simulink model "single_phase_multilevel_sm"  (R2026a)
settings: Solver=ode1be  StopTime=simlength  FixedStep=tc
values from neighbouring files (symbols this model uses):
  Vfc1_base = Udc/5    [plotting_modulation.m]    (also in plotting_results.m; plotting_results_hf.m)
  Vfc2_base = 2*Vfc1_base    [plotting_modulation.m]    (also in plotting_results.m; plotting_results_hf.m)
  Vfc3_base = 3*Vfc1_base    [plotting_modulation.m]    (also in plotting_results.m; plotting_results_hf.m)
  Vfc4_base = 4*Vfc1_base    [plotting_modulation.m]    (also in plotting_results.m; plotting_results_hf.m)
undefined symbols (not defined in the file or in its folder): g0_4Hz, g1_4Hz, I_FS, kalman_omega, kalman_theta, ki_i_inv, ki_v_inv, kp_i_inv, kp_v_inv, Lconn, LFu1, m_dead_time, m_duty_open_loop, magnitude, n1, n10, omega_ref, phase_shift_mod11, phase_shift_mod21, phase_shift_mod31, phase_shift_mod41, phase_shift_mod51, precharge_off, q1kalman, q2kalman, Rbalance, Rconn, RFu, Rkalman, RLFu1, tc, time_pwm_enable, tPWM, ts, V_FS, VCFc_5_init, Vgate_base
libraries: fl_lib x103, nesl_utility x61, simulink x1
(part 2 of 3)

== system single_phase_multilevel_sm/flying_capacitor_leg/fc1 ==
  CFc_1 : fl_lib/Electrical/Electrical Elements/Capacitor  c=CFc_1 F  r=1e-6 Ohm  g=0 1/Ohm  i_specify=off  i_priority=None  i=0 A  i_nominal_specify=off  i_nominal_value=1  i_nominal_unit=A  v_specify=off  v_priority=None  v=0 V  v_nominal_specify=off  v_nominal_value=1  v_nominal_unit=V  vc_specify=on  vc_priority=High  vc=VCFc_1_init V  vc_nominal_specify=off  vc_nominal_value=1  vc_nominal_unit=V
  CFi_HF_1 : fl_lib/Electrical/Electrical Elements/Capacitor  c=CFi_HF_1 F  r=1e-6 Ohm  g=0 1/Ohm  i_specify=off  i_priority=None  i=0 A  i_nominal_specify=off  i_nominal_value=1  i_nominal_unit=A  v_specify=off  v_priority=None  v=0 V  v_nominal_specify=off  v_nominal_value=1  v_nominal_unit=V  vc_specify=on  vc_priority=High  vc=VCFc_1_init V  vc_nominal_specify=off  vc_nominal_value=1  vc_nominal_unit=V
  Current Sensor : fl_lib/Electrical/Electrical Sensors/Current Sensor
  Current Sensor1 : fl_lib/Electrical/Electrical Sensors/Current Sensor
  PS-Simulink Converter : nesl_utility/PS-Simulink Converter  PhysicalDomain=network_engine_domain  SubClassName=ps_output  LeftPortType=input  RightPortType=output  PseudoPeriodic=off  Frequencies=[]  VectorFormat=1-D array  Unit=A  AffineConversion=off
  PS-Simulink Converter1 : nesl_utility/PS-Simulink Converter  PhysicalDomain=network_engine_domain  SubClassName=ps_output  LeftPortType=input  RightPortType=output  PseudoPeriodic=off  Frequencies=[]  VectorFormat=1-D array  Unit=V  AffineConversion=off
  PS-Simulink Converter2 : nesl_utility/PS-Simulink Converter  PhysicalDomain=network_engine_domain  SubClassName=ps_output  LeftPortType=input  RightPortType=output  PseudoPeriodic=off  Frequencies=[]  VectorFormat=1-D array  Unit=A  AffineConversion=off
  Voltage Sensor : fl_lib/Electrical/Electrical Sensors/Voltage Sensor
  1 : PMIOPort  Side=Left
  2 : PMIOPort  Port=2  Side=Right
  tag scope: current_flying_capacitor_1=global, current_hf_capacitor_1=global, voltage_flying_capacitor_1=global
  wires:
  PS-Simulink Converter1/1 -> [voltage_flying_capacitor_1]
  PS-Simulink Converter/1 -> [current_flying_capacitor_1]
  PS-Simulink Converter2/1 -> [current_hf_capacitor_1]
  connections:
  Current Sensor/RConn2 -- CFc_1/LConn1
  Voltage Sensor/RConn1 -- PS-Simulink Converter1/LConn1
  Current Sensor/RConn1 -- PS-Simulink Converter/LConn1
  Current Sensor/LConn1 -- Current Sensor1/LConn1 -- 1/RConn1 -- Voltage Sensor/LConn1
  Voltage Sensor/RConn2 -- 2/RConn1 -- CFc_1/RConn1 -- CFi_HF_1/RConn1
  Current Sensor1/RConn2 -- CFi_HF_1/LConn1
  Current Sensor1/RConn1 -- PS-Simulink Converter2/LConn1

== system single_phase_multilevel_sm/flying_capacitor_leg/fc2 ==
  CFc_2 : fl_lib/Electrical/Electrical Elements/Capacitor  c=CFc_2 F  r=1e-6 Ohm  g=0 1/Ohm  i_specify=off  i_priority=None  i=0 A  i_nominal_specify=off  i_nominal_value=1  i_nominal_unit=A  v_specify=off  v_priority=None  v=0 V  v_nominal_specify=off  v_nominal_value=1  v_nominal_unit=V  vc_specify=on  vc_priority=High  vc=VCFc_2_init V  vc_nominal_specify=off  vc_nominal_value=1  vc_nominal_unit=V
  CFi_HF_2 : fl_lib/Electrical/Electrical Elements/Capacitor  c=CFi_HF_2 F  r=1e-6 Ohm  g=0 1/Ohm  i_specify=off  i_priority=None  i=0 A  i_nominal_specify=off  i_nominal_value=1  i_nominal_unit=A  v_specify=off  v_priority=None  v=0 V  v_nominal_specify=off  v_nominal_value=1  v_nominal_unit=V  vc_specify=on  vc_priority=High  vc=VCFc_2_init V  vc_nominal_specify=off  vc_nominal_value=1  vc_nominal_unit=V
  Current Sensor : fl_lib/Electrical/Electrical Sensors/Current Sensor
  PS-Simulink Converter : nesl_utility/PS-Simulink Converter  PhysicalDomain=network_engine_domain  SubClassName=ps_output  LeftPortType=input  RightPortType=output  PseudoPeriodic=off  Frequencies=[]  VectorFormat=1-D array  Unit=A  AffineConversion=off
  PS-Simulink Converter2 : nesl_utility/PS-Simulink Converter  PhysicalDomain=network_engine_domain  SubClassName=ps_output  LeftPortType=input  RightPortType=output  PseudoPeriodic=off  Frequencies=[]  VectorFormat=1-D array  Unit=V  AffineConversion=off
  Voltage Sensor1 : fl_lib/Electrical/Electrical Sensors/Voltage Sensor
  1 : PMIOPort  Side=Left
  2 : PMIOPort  Port=2  Side=Right
  tag scope: current_flying_capacitor_2=global, voltage_flying_capacitor_2=global
  wires:
  PS-Simulink Converter2/1 -> [voltage_flying_capacitor_2]
  PS-Simulink Converter/1 -> [current_flying_capacitor_2]
  connections:
  Voltage Sensor1/LConn1 -- CFi_HF_2/LConn1 -- CFc_2/LConn1 -- 1/RConn1
  Voltage Sensor1/RConn1 -- PS-Simulink Converter2/LConn1
  Current Sensor/RConn1 -- PS-Simulink Converter/LConn1
  CFc_2/RConn1 -- Current Sensor/LConn1
  Voltage Sensor1/RConn2 -- CFi_HF_2/RConn1 -- Current Sensor/RConn2 -- 2/RConn1

== system single_phase_multilevel_sm/flying_capacitor_leg/fc3 ==
  CFc_3 : fl_lib/Electrical/Electrical Elements/Capacitor  c=CFc_3 F  r=1e-6 Ohm  g=0 1/Ohm  i_specify=off  i_priority=None  i=0 A  i_nominal_specify=off  i_nominal_value=1  i_nominal_unit=A  v_specify=off  v_priority=None  v=0 V  v_nominal_specify=off  v_nominal_value=1  v_nominal_unit=V  vc_specify=on  vc_priority=High  vc=VCFc_3_init V  vc_nominal_specify=off  vc_nominal_value=1  vc_nominal_unit=V
  CFi_HF_3 : fl_lib/Electrical/Electrical Elements/Capacitor  c=CFi_HF_3 F  r=1e-6 Ohm  g=0 1/Ohm  i_specify=off  i_priority=None  i=0 A  i_nominal_specify=off  i_nominal_value=1  i_nominal_unit=A  v_specify=off  v_priority=None  v=0 V  v_nominal_specify=off  v_nominal_value=1  v_nominal_unit=V  vc_specify=on  vc_priority=High  vc=VCFc_3_init V  vc_nominal_specify=off  vc_nominal_value=1  vc_nominal_unit=V
  Current Sensor : fl_lib/Electrical/Electrical Sensors/Current Sensor
  PS-Simulink Converter : nesl_utility/PS-Simulink Converter  PhysicalDomain=network_engine_domain  SubClassName=ps_output  LeftPortType=input  RightPortType=output  PseudoPeriodic=off  Frequencies=[]  VectorFormat=1-D array  Unit=A  AffineConversion=off
  PS-Simulink Converter2 : nesl_utility/PS-Simulink Converter  PhysicalDomain=network_engine_domain  SubClassName=ps_output  LeftPortType=input  RightPortType=output  PseudoPeriodic=off  Frequencies=[]  VectorFormat=1-D array  Unit=V  AffineConversion=off
  Voltage Sensor1 : fl_lib/Electrical/Electrical Sensors/Voltage Sensor
  1 : PMIOPort  Side=Left
  2 : PMIOPort  Port=2  Side=Right
  tag scope: current_flying_capacitor_3=global, voltage_flying_capacitor_3=global
  wires:
  PS-Simulink Converter2/1 -> [voltage_flying_capacitor_3]
  PS-Simulink Converter/1 -> [current_flying_capacitor_3]
  connections:
  CFc_3/LConn1 -- CFi_HF_3/LConn1 -- Voltage Sensor1/LConn1 -- 1/RConn1
  Voltage Sensor1/RConn1 -- PS-Simulink Converter2/LConn1
  Voltage Sensor1/RConn2 -- CFi_HF_3/RConn1 -- Current Sensor/RConn2 -- 2/RConn1
  Current Sensor/RConn1 -- PS-Simulink Converter/LConn1
  Current Sensor/LConn1 -- CFc_3/RConn1

== system single_phase_multilevel_sm/flying_capacitor_leg/fc4 ==
  CFc_4 : fl_lib/Electrical/Electrical Elements/Capacitor  c=CFc_4 F  r=1e-6 Ohm  g=0 1/Ohm  i_specify=off  i_priority=None  i=0 A  i_nominal_specify=off  i_nominal_value=1  i_nominal_unit=A  v_specify=off  v_priority=None  v=0 V  v_nominal_specify=off  v_nominal_value=1  v_nominal_unit=V  vc_specify=on  vc_priority=High  vc=VCFc_4_init V  vc_nominal_specify=off  vc_nominal_value=1  vc_nominal_unit=V
  CFi_HF_4 : fl_lib/Electrical/Electrical Elements/Capacitor  c=CFi_HF_4 F  r=1e-6 Ohm  g=0 1/Ohm  i_specify=off  i_priority=None  i=0 A  i_nominal_specify=off  i_nominal_value=1  i_nominal_unit=A  v_specify=off  v_priority=None  v=0 V  v_nominal_specify=off  v_nominal_value=1  v_nominal_unit=V  vc_specify=on  vc_priority=High  vc=VCFc_4_init V  vc_nominal_specify=off  vc_nominal_value=1  vc_nominal_unit=V
  Current Sensor : fl_lib/Electrical/Electrical Sensors/Current Sensor
  PS-Simulink Converter : nesl_utility/PS-Simulink Converter  PhysicalDomain=network_engine_domain  SubClassName=ps_output  LeftPortType=input  RightPortType=output  PseudoPeriodic=off  Frequencies=[]  VectorFormat=1-D array  Unit=A  AffineConversion=off
  PS-Simulink Converter2 : nesl_utility/PS-Simulink Converter  PhysicalDomain=network_engine_domain  SubClassName=ps_output  LeftPortType=input  RightPortType=output  PseudoPeriodic=off  Frequencies=[]  VectorFormat=1-D array  Unit=V  AffineConversion=off
  Voltage Sensor1 : fl_lib/Electrical/Electrical Sensors/Voltage Sensor
  1 : PMIOPort  Side=Left
  2 : PMIOPort  Port=2  Side=Right
  tag scope: current_flying_capacitor_4=global, voltage_flying_capacitor_4=global
  wires:
  PS-Simulink Converter2/1 -> [voltage_flying_capacitor_4]
  PS-Simulink Converter/1 -> [current_flying_capacitor_4]
  connections:
  Voltage Sensor1/LConn1 -- CFi_HF_4/LConn1 -- CFc_4/LConn1 -- 1/RConn1
  Voltage Sensor1/RConn1 -- PS-Simulink Converter2/LConn1
  Voltage Sensor1/RConn2 -- CFi_HF_4/RConn1 -- Current Sensor/RConn2 -- 2/RConn1
  Current Sensor/RConn1 -- PS-Simulink Converter/LConn1
  Current Sensor/LConn1 -- CFc_4/RConn1

== system single_phase_multilevel_sm/flying_capacitor_leg/fc51 ==
  CFc_51 : fl_lib/Electrical/Electrical Elements/Capacitor  c=CFc_51 F  r=1e-6 Ohm  g=0 1/Ohm  i_specify=off  i_priority=None  i=0 A  i_nominal_specify=off  i_nominal_value=1  i_nominal_unit=A  v_specify=off  v_priority=None  v=0 V  v_nominal_specify=off  v_nominal_value=1  v_nominal_unit=V  vc_specify=on  vc_priority=High  vc=VCFc_5_init/2 V  vc_nominal_specify=off  vc_nominal_value=1  vc_nominal_unit=V
  Current Sensor : fl_lib/Electrical/Electrical Sensors/Current Sensor
  PS-Simulink Converter : nesl_utility/PS-Simulink Converter  PhysicalDomain=network_engine_domain  SubClassName=ps_output  LeftPortType=input  RightPortType=output  PseudoPeriodic=off  Frequencies=[]  VectorFormat=1-D array  Unit=A  AffineConversion=off
  PS-Simulink Converter2 : nesl_utility/PS-Simulink Converter  PhysicalDomain=network_engine_domain  SubClassName=ps_output  LeftPortType=input  RightPortType=output  PseudoPeriodic=off  Frequencies=[]  VectorFormat=1-D array  Unit=V  AffineConversion=off
  Voltage Sensor1 : fl_lib/Electrical/Electrical Sensors/Voltage Sensor
  1 : PMIOPort  Side=Left
  2 : PMIOPort  Port=2  Side=Right
  tag scope: current_flying_capacitor_51=global, voltage_flying_capacitor_51=global
  wires:
  PS-Simulink Converter/1 -> [current_flying_capacitor_51]
  PS-Simulink Converter2/1 -> [voltage_flying_capacitor_51]
  connections:
  CFc_51/LConn1 -- Voltage Sensor1/LConn1 -- 1/RConn1
  Current Sensor/RConn1 -- PS-Simulink Converter/LConn1
  Current Sensor/LConn1 -- CFc_51/RConn1
  Current Sensor/RConn2 -- Voltage Sensor1/RConn2 -- 2/RConn1
  Voltage Sensor1/RConn1 -- PS-Simulink Converter2/LConn1

== system single_phase_multilevel_sm/flying_capacitor_leg/fc52 ==
  CFc_52 : fl_lib/Electrical/Electrical Elements/Capacitor  c=CFc_52 F  r=1e-6 Ohm  g=0 1/Ohm  i_specify=off  i_priority=None  i=0 A  i_nominal_specify=off  i_nominal_value=1  i_nominal_unit=A  v_specify=off  v_priority=None  v=0 V  v_nominal_specify=off  v_nominal_value=1  v_nominal_unit=V  vc_specify=on  vc_priority=High  vc=VCFc_5_init/2 V  vc_nominal_specify=off  vc_nominal_value=1  vc_nominal_unit=V
  Current Sensor : fl_lib/Electrical/Electrical Sensors/Current Sensor
  PS-Simulink Converter : nesl_utility/PS-Simulink Converter  PhysicalDomain=network_engine_domain  SubClassName=ps_output  LeftPortType=input  RightPortType=output  PseudoPeriodic=off  Frequencies=[]  VectorFormat=1-D array  Unit=A  AffineConversion=off
  PS-Simulink Converter2 : nesl_utility/PS-Simulink Converter  PhysicalDomain=network_engine_domain  SubClassName=ps_output  LeftPortType=input  RightPortType=output  PseudoPeriodic=off  Frequencies=[]  VectorFormat=1-D array  Unit=V  AffineConversion=off
  Voltage Sensor1 : fl_lib/Electrical/Electrical Sensors/Voltage Sensor
  1 : PMIOPort  Side=Left
  2 : PMIOPort  Port=2  Side=Right
  tag scope: current_flying_capacitor_52=global, voltage_flying_capacitor_52=global
  wires:
  PS-Simulink Converter/1 -> [current_flying_capacitor_52]
  PS-Simulink Converter2/1 -> [voltage_flying_capacitor_52]
  connections:
  CFc_52/LConn1 -- Voltage Sensor1/LConn1 -- 1/RConn1
  Current Sensor/RConn1 -- PS-Simulink Converter/LConn1
  Current Sensor/RConn2 -- Voltage Sensor1/RConn2 -- 2/RConn1
  CFc_52/RConn1 -- Current Sensor/LConn1
  Voltage Sensor1/RConn1 -- PS-Simulink Converter2/LConn1

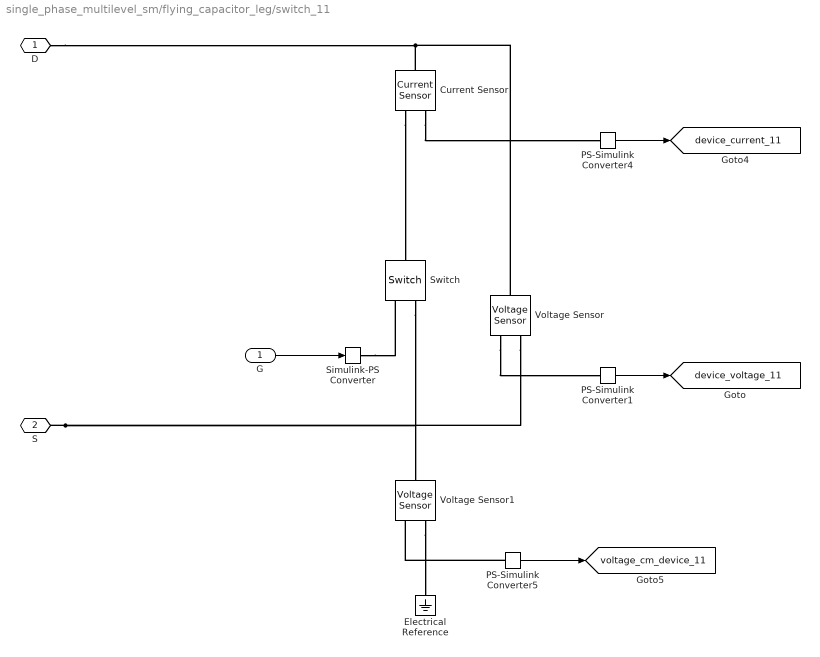
== system single_phase_multilevel_sm/flying_capacitor_leg/switch_11 ==
  G : Inport
  Current Sensor : fl_lib/Electrical/Electrical Sensors/Current Sensor
  Electrical Reference : fl_lib/Electrical/Electrical Elements/Electrical Reference
  PS-Simulink Converter1 : nesl_utility/PS-Simulink Converter  PhysicalDomain=network_engine_domain  SubClassName=ps_output  LeftPortType=input  RightPortType=output  PseudoPeriodic=off  Frequencies=[]  VectorFormat=1-D array  Unit=V  AffineConversion=off
  PS-Simulink Converter4 : nesl_utility/PS-Simulink Converter  PhysicalDomain=network_engine_domain  SubClassName=ps_output  LeftPortType=input  RightPortType=output  PseudoPeriodic=off  Frequencies=[]  VectorFormat=1-D array  Unit=A  AffineConversion=off
  PS-Simulink Converter5 : nesl_utility/PS-Simulink Converter  PhysicalDomain=network_engine_domain  SubClassName=ps_output  LeftPortType=input  RightPortType=output  PseudoPeriodic=off  Frequencies=[]  VectorFormat=1-D array  Unit=V  AffineConversion=off
  Simulink-PS Converter : nesl_utility/Simulink-PS Converter  PhysicalDomain=network_engine_domain  SubClassName=ps_input  LeftPortType=input  RightPortType=output  PseudoPeriodic=off  Frequencies=[]  NoiseDistribution=none  NoiseParameters=[]  Unit=V  AffineConversion=off  FilteringAndDerivatives=provide  SimscapeFilterOrder=1  InputFilterTimeConstant=0.001  UdotUserProvided=0
  Switch : fl_lib/Electrical/Electrical Elements/Switch  R_closed=1e-3 Ohm  G_open=1e-8 1/Ohm  Threshold=3  i_specify=off  i_priority=None  i=0 A  i_nominal_specify=off  i_nominal_value=1  i_nominal_unit=A  v_specify=off  v_priority=None  v=0 V  v_nominal_specify=off  v_nominal_value=1  v_nominal_unit=V
  Voltage Sensor : fl_lib/Electrical/Electrical Sensors/Voltage Sensor
  Voltage Sensor1 : fl_lib/Electrical/Electrical Sensors/Voltage Sensor
  D : PMIOPort  Side=Left
  S : PMIOPort  Port=2  Side=Right
  tag scope: device_current_11=global, device_voltage_11=global, voltage_cm_device_11=global
  wires:
  PS-Simulink Converter1/1 -> [device_voltage_11]
  PS-Simulink Converter4/1 -> [device_current_11]
  PS-Simulink Converter5/1 -> [voltage_cm_device_11]
  G/1 -> Simulink-PS Converter/1
  connections:
  Voltage Sensor/RConn1 -- PS-Simulink Converter1/LConn1
  S/RConn1 -- Switch/RConn2 -- Voltage Sensor/RConn2 -- Voltage Sensor1/LConn1
  Current Sensor/LConn1 -- D/RConn1 -- Voltage Sensor/LConn1
  Current Sensor/RConn1 -- PS-Simulink Converter4/LConn1
  PS-Simulink Converter5/LConn1 -- Voltage Sensor1/RConn1
  Voltage Sensor1/RConn2 -- Electrical Reference/LConn1
  Simulink-PS Converter/RConn1 -- Switch/RConn1
  Current Sensor/RConn2 -- Switch/LConn1

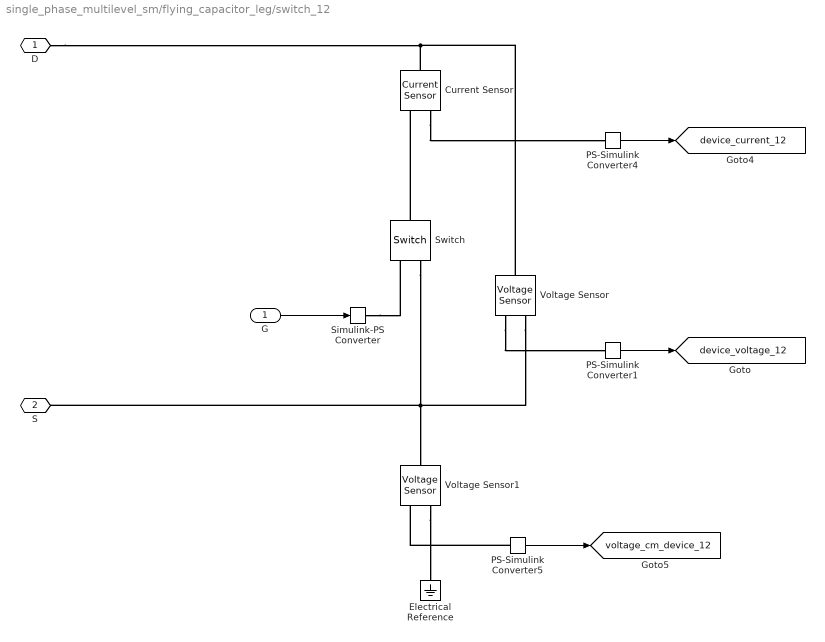
== system single_phase_multilevel_sm/flying_capacitor_leg/switch_12 ==
  G : Inport
  Current Sensor : fl_lib/Electrical/Electrical Sensors/Current Sensor
  Electrical Reference : fl_lib/Electrical/Electrical Elements/Electrical Reference
  PS-Simulink Converter1 : nesl_utility/PS-Simulink Converter  PhysicalDomain=network_engine_domain  SubClassName=ps_output  LeftPortType=input  RightPortType=output  PseudoPeriodic=off  Frequencies=[]  VectorFormat=1-D array  Unit=V  AffineConversion=off
  PS-Simulink Converter4 : nesl_utility/PS-Simulink Converter  PhysicalDomain=network_engine_domain  SubClassName=ps_output  LeftPortType=input  RightPortType=output  PseudoPeriodic=off  Frequencies=[]  VectorFormat=1-D array  Unit=A  AffineConversion=off
  PS-Simulink Converter5 : nesl_utility/PS-Simulink Converter  PhysicalDomain=network_engine_domain  SubClassName=ps_output  LeftPortType=input  RightPortType=output  PseudoPeriodic=off  Frequencies=[]  VectorFormat=1-D array  Unit=V  AffineConversion=off
  Simulink-PS Converter : nesl_utility/Simulink-PS Converter  PhysicalDomain=network_engine_domain  SubClassName=ps_input  LeftPortType=input  RightPortType=output  PseudoPeriodic=off  Frequencies=[]  NoiseDistribution=none  NoiseParameters=[]  Unit=V  AffineConversion=off  FilteringAndDerivatives=provide  SimscapeFilterOrder=1  InputFilterTimeConstant=0.001  UdotUserProvided=0
  Switch : fl_lib/Electrical/Electrical Elements/Switch  R_closed=1e-3 Ohm  G_open=1e-8 1/Ohm  Threshold=3  i_specify=off  i_priority=None  i=0 A  i_nominal_specify=off  i_nominal_value=1  i_nominal_unit=A  v_specify=off  v_priority=None  v=0 V  v_nominal_specify=off  v_nominal_value=1  v_nominal_unit=V
  Voltage Sensor : fl_lib/Electrical/Electrical Sensors/Voltage Sensor
  Voltage Sensor1 : fl_lib/Electrical/Electrical Sensors/Voltage Sensor
  D : PMIOPort  Side=Left
  S : PMIOPort  Port=2  Side=Right
  tag scope: device_current_12=global, device_voltage_12=global, voltage_cm_device_12=global
  wires:
  PS-Simulink Converter1/1 -> [device_voltage_12]
  PS-Simulink Converter4/1 -> [device_current_12]
  PS-Simulink Converter5/1 -> [voltage_cm_device_12]
  G/1 -> Simulink-PS Converter/1
  connections:
  Voltage Sensor/RConn2 -- S/RConn1 -- Switch/RConn2 -- Voltage Sensor1/LConn1
  Voltage Sensor/RConn1 -- PS-Simulink Converter1/LConn1
  Current Sensor/LConn1 -- D/RConn1 -- Voltage Sensor/LConn1
  Current Sensor/RConn1 -- PS-Simulink Converter4/LConn1
  PS-Simulink Converter5/LConn1 -- Voltage Sensor1/RConn1
  Voltage Sensor1/RConn2 -- Electrical Reference/LConn1
  Simulink-PS Converter/RConn1 -- Switch/RConn1
  Switch/LConn1 -- Current Sensor/RConn2

== system single_phase_multilevel_sm/flying_capacitor_leg/switch_21 ==
  G : Inport
  Current Sensor : fl_lib/Electrical/Electrical Sensors/Current Sensor
  Electrical Reference : fl_lib/Electrical/Electrical Elements/Electrical Reference
  PS-Simulink Converter1 : nesl_utility/PS-Simulink Converter  PhysicalDomain=network_engine_domain  SubClassName=ps_output  LeftPortType=input  RightPortType=output  PseudoPeriodic=off  Frequencies=[]  VectorFormat=1-D array  Unit=V  AffineConversion=off
  PS-Simulink Converter4 : nesl_utility/PS-Simulink Converter  PhysicalDomain=network_engine_domain  SubClassName=ps_output  LeftPortType=input  RightPortType=output  PseudoPeriodic=off  Frequencies=[]  VectorFormat=1-D array  Unit=A  AffineConversion=off
  PS-Simulink Converter5 : nesl_utility/PS-Simulink Converter  PhysicalDomain=network_engine_domain  SubClassName=ps_output  LeftPortType=input  RightPortType=output  PseudoPeriodic=off  Frequencies=[]  VectorFormat=1-D array  Unit=V  AffineConversion=off
  Simulink-PS Converter : nesl_utility/Simulink-PS Converter  PhysicalDomain=network_engine_domain  SubClassName=ps_input  LeftPortType=input  RightPortType=output  PseudoPeriodic=off  Frequencies=[]  NoiseDistribution=none  NoiseParameters=[]  Unit=V  AffineConversion=off  FilteringAndDerivatives=provide  SimscapeFilterOrder=1  InputFilterTimeConstant=0.001  UdotUserProvided=0
  Switch : fl_lib/Electrical/Electrical Elements/Switch  R_closed=1e-3 Ohm  G_open=1e-8 1/Ohm  Threshold=3  i_specify=off  i_priority=None  i=0 A  i_nominal_specify=off  i_nominal_value=1  i_nominal_unit=A  v_specify=off  v_priority=None  v=0 V  v_nominal_specify=off  v_nominal_value=1  v_nominal_unit=V
  Voltage Sensor : fl_lib/Electrical/Electrical Sensors/Voltage Sensor
  Voltage Sensor1 : fl_lib/Electrical/Electrical Sensors/Voltage Sensor
  D : PMIOPort  Side=Left
  S : PMIOPort  Port=2  Side=Right
  tag scope: device_current_21=global, device_voltage_21=global, voltage_cm_device_21=global
  wires:
  PS-Simulink Converter1/1 -> [device_voltage_21]
  PS-Simulink Converter4/1 -> [device_current_21]
  PS-Simulink Converter5/1 -> [voltage_cm_device_21]
  G/1 -> Simulink-PS Converter/1
  connections:
  Voltage Sensor/RConn2 -- Switch/RConn2 -- S/RConn1 -- Voltage Sensor1/LConn1
  Voltage Sensor/RConn1 -- PS-Simulink Converter1/LConn1
  Current Sensor/LConn1 -- Voltage Sensor/LConn1 -- D/RConn1
  Current Sensor/RConn1 -- PS-Simulink Converter4/LConn1
  PS-Simulink Converter5/LConn1 -- Voltage Sensor1/RConn1
  Voltage Sensor1/RConn2 -- Electrical Reference/LConn1
  Simulink-PS Converter/RConn1 -- Switch/RConn1
  Current Sensor/RConn2 -- Switch/LConn1

== system single_phase_multilevel_sm/flying_capacitor_leg/switch_22 ==
  G : Inport
  Current Sensor : fl_lib/Electrical/Electrical Sensors/Current Sensor
  Electrical Reference : fl_lib/Electrical/Electrical Elements/Electrical Reference
  PS-Simulink Converter1 : nesl_utility/PS-Simulink Converter  PhysicalDomain=network_engine_domain  SubClassName=ps_output  LeftPortType=input  RightPortType=output  PseudoPeriodic=off  Frequencies=[]  VectorFormat=1-D array  Unit=V  AffineConversion=off
  PS-Simulink Converter4 : nesl_utility/PS-Simulink Converter  PhysicalDomain=network_engine_domain  SubClassName=ps_output  LeftPortType=input  RightPortType=output  PseudoPeriodic=off  Frequencies=[]  VectorFormat=1-D array  Unit=A  AffineConversion=off
  PS-Simulink Converter5 : nesl_utility/PS-Simulink Converter  PhysicalDomain=network_engine_domain  SubClassName=ps_output  LeftPortType=input  RightPortType=output  PseudoPeriodic=off  Frequencies=[]  VectorFormat=1-D array  Unit=V  AffineConversion=off
  Simulink-PS Converter : nesl_utility/Simulink-PS Converter  PhysicalDomain=network_engine_domain  SubClassName=ps_input  LeftPortType=input  RightPortType=output  PseudoPeriodic=off  Frequencies=[]  NoiseDistribution=none  NoiseParameters=[]  Unit=V  AffineConversion=off  FilteringAndDerivatives=provide  SimscapeFilterOrder=1  InputFilterTimeConstant=0.001  UdotUserProvided=0
  Switch : fl_lib/Electrical/Electrical Elements/Switch  R_closed=1e-3 Ohm  G_open=1e-8 1/Ohm  Threshold=3  i_specify=off  i_priority=None  i=0 A  i_nominal_specify=off  i_nominal_value=1  i_nominal_unit=A  v_specify=off  v_priority=None  v=0 V  v_nominal_specify=off  v_nominal_value=1  v_nominal_unit=V
  Voltage Sensor : fl_lib/Electrical/Electrical Sensors/Voltage Sensor
  Voltage Sensor1 : fl_lib/Electrical/Electrical Sensors/Voltage Sensor
  D : PMIOPort  Side=Left
  S : PMIOPort  Port=2  Side=Right
  tag scope: device_current_22=global, device_voltage_22=global, voltage_cm_device_22=global
  wires:
  PS-Simulink Converter1/1 -> [device_voltage_22]
  PS-Simulink Converter4/1 -> [device_current_22]
  PS-Simulink Converter5/1 -> [voltage_cm_device_22]
  G/1 -> Simulink-PS Converter/1
  connections:
  Voltage Sensor/RConn1 -- PS-Simulink Converter1/LConn1
  S/RConn1 -- Switch/RConn2 -- Voltage Sensor/RConn2 -- Voltage Sensor1/LConn1
  Current Sensor/LConn1 -- Voltage Sensor/LConn1 -- D/RConn1
  Current Sensor/RConn1 -- PS-Simulink Converter4/LConn1
  PS-Simulink Converter5/LConn1 -- Voltage Sensor1/RConn1
  Voltage Sensor1/RConn2 -- Electrical Reference/LConn1
  Simulink-PS Converter/RConn1 -- Switch/RConn1
  Switch/LConn1 -- Current Sensor/RConn2

== system single_phase_multilevel_sm/flying_capacitor_leg/switch_31 ==
  G : Inport
  Current Sensor : fl_lib/Electrical/Electrical Sensors/Current Sensor
  Electrical Reference : fl_lib/Electrical/Electrical Elements/Electrical Reference
  PS-Simulink Converter1 : nesl_utility/PS-Simulink Converter  PhysicalDomain=network_engine_domain  SubClassName=ps_output  LeftPortType=input  RightPortType=output  PseudoPeriodic=off  Frequencies=[]  VectorFormat=1-D array  Unit=V  AffineConversion=off
  PS-Simulink Converter4 : nesl_utility/PS-Simulink Converter  PhysicalDomain=network_engine_domain  SubClassName=ps_output  LeftPortType=input  RightPortType=output  PseudoPeriodic=off  Frequencies=[]  VectorFormat=1-D array  Unit=A  AffineConversion=off
  PS-Simulink Converter5 : nesl_utility/PS-Simulink Converter  PhysicalDomain=network_engine_domain  SubClassName=ps_output  LeftPortType=input  RightPortType=output  PseudoPeriodic=off  Frequencies=[]  VectorFormat=1-D array  Unit=V  AffineConversion=off
  Simulink-PS Converter : nesl_utility/Simulink-PS Converter  PhysicalDomain=network_engine_domain  SubClassName=ps_input  LeftPortType=input  RightPortType=output  PseudoPeriodic=off  Frequencies=[]  NoiseDistribution=none  NoiseParameters=[]  Unit=V  AffineConversion=off  FilteringAndDerivatives=provide  SimscapeFilterOrder=1  InputFilterTimeConstant=0.001  UdotUserProvided=0
  Switch : fl_lib/Electrical/Electrical Elements/Switch  R_closed=1e-3 Ohm  G_open=1e-8 1/Ohm  Threshold=3  i_specify=off  i_priority=None  i=0 A  i_nominal_specify=off  i_nominal_value=1  i_nominal_unit=A  v_specify=off  v_priority=None  v=0 V  v_nominal_specify=off  v_nominal_value=1  v_nominal_unit=V
  Voltage Sensor : fl_lib/Electrical/Electrical Sensors/Voltage Sensor
  Voltage Sensor1 : fl_lib/Electrical/Electrical Sensors/Voltage Sensor
  D : PMIOPort  Side=Left
  S : PMIOPort  Port=2  Side=Right
  tag scope: device_current_31=global, device_voltage_31=global, voltage_cm_device_31=global
  wires:
  PS-Simulink Converter1/1 -> [device_voltage_31]
  PS-Simulink Converter4/1 -> [device_current_31]
  PS-Simulink Converter5/1 -> [voltage_cm_device_31]
  G/1 -> Simulink-PS Converter/1
  connections:
  Voltage Sensor/RConn1 -- PS-Simulink Converter1/LConn1
  S/RConn1 -- Switch/RConn2 -- Voltage Sensor/RConn2 -- Voltage Sensor1/LConn1
  Current Sensor/LConn1 -- Voltage Sensor/LConn1 -- D/RConn1
  Current Sensor/RConn1 -- PS-Simulink Converter4/LConn1
  PS-Simulink Converter5/LConn1 -- Voltage Sensor1/RConn1
  Voltage Sensor1/RConn2 -- Electrical Reference/LConn1
  Simulink-PS Converter/RConn1 -- Switch/RConn1
  Current Sensor/RConn2 -- Switch/LConn1

== system single_phase_multilevel_sm/flying_capacitor_leg/switch_32 ==
  G : Inport
  Current Sensor : fl_lib/Electrical/Electrical Sensors/Current Sensor
  Electrical Reference : fl_lib/Electrical/Electrical Elements/Electrical Reference
  PS-Simulink Converter1 : nesl_utility/PS-Simulink Converter  PhysicalDomain=network_engine_domain  SubClassName=ps_output  LeftPortType=input  RightPortType=output  PseudoPeriodic=off  Frequencies=[]  VectorFormat=1-D array  Unit=V  AffineConversion=off
  PS-Simulink Converter4 : nesl_utility/PS-Simulink Converter  PhysicalDomain=network_engine_domain  SubClassName=ps_output  LeftPortType=input  RightPortType=output  PseudoPeriodic=off  Frequencies=[]  VectorFormat=1-D array  Unit=A  AffineConversion=off
  PS-Simulink Converter5 : nesl_utility/PS-Simulink Converter  PhysicalDomain=network_engine_domain  SubClassName=ps_output  LeftPortType=input  RightPortType=output  PseudoPeriodic=off  Frequencies=[]  VectorFormat=1-D array  Unit=V  AffineConversion=off
  Simulink-PS Converter : nesl_utility/Simulink-PS Converter  PhysicalDomain=network_engine_domain  SubClassName=ps_input  LeftPortType=input  RightPortType=output  PseudoPeriodic=off  Frequencies=[]  NoiseDistribution=none  NoiseParameters=[]  Unit=V  AffineConversion=off  FilteringAndDerivatives=provide  SimscapeFilterOrder=1  InputFilterTimeConstant=0.001  UdotUserProvided=0
  Switch : fl_lib/Electrical/Electrical Elements/Switch  R_closed=1e-3 Ohm  G_open=1e-8 1/Ohm  Threshold=3  i_specify=off  i_priority=None  i=0 A  i_nominal_specify=off  i_nominal_value=1  i_nominal_unit=A  v_specify=off  v_priority=None  v=0 V  v_nominal_specify=off  v_nominal_value=1  v_nominal_unit=V
  Voltage Sensor : fl_lib/Electrical/Electrical Sensors/Voltage Sensor
  Voltage Sensor1 : fl_lib/Electrical/Electrical Sensors/Voltage Sensor
  D : PMIOPort  Side=Left
  S : PMIOPort  Port=2  Side=Right
  tag scope: device_current_32=global, device_voltage_32=global, voltage_cm_device_32=global
  wires:
  PS-Simulink Converter1/1 -> [device_voltage_32]
  PS-Simulink Converter4/1 -> [device_current_32]
  PS-Simulink Converter5/1 -> [voltage_cm_device_32]
  G/1 -> Simulink-PS Converter/1
  connections:
  Voltage Sensor/RConn2 -- Voltage Sensor1/LConn1 -- Switch/RConn2 -- S/RConn1
  Voltage Sensor/RConn1 -- PS-Simulink Converter1/LConn1
  Current Sensor/LConn1 -- D/RConn1 -- Voltage Sensor/LConn1
  Current Sensor/RConn1 -- PS-Simulink Converter4/LConn1
  PS-Simulink Converter5/LConn1 -- Voltage Sensor1/RConn1
  Voltage Sensor1/RConn2 -- Electrical Reference/LConn1
  Simulink-PS Converter/RConn1 -- Switch/RConn1
  Switch/LConn1 -- Current Sensor/RConn2

== system single_phase_multilevel_sm/flying_capacitor_leg/switch_41 ==
  G : Inport
  Current Sensor : fl_lib/Electrical/Electrical Sensors/Current Sensor
  Electrical Reference : fl_lib/Electrical/Electrical Elements/Electrical Reference
  PS-Simulink Converter1 : nesl_utility/PS-Simulink Converter  PhysicalDomain=network_engine_domain  SubClassName=ps_output  LeftPortType=input  RightPortType=output  PseudoPeriodic=off  Frequencies=[]  VectorFormat=1-D array  Unit=V  AffineConversion=off
  PS-Simulink Converter4 : nesl_utility/PS-Simulink Converter  PhysicalDomain=network_engine_domain  SubClassName=ps_output  LeftPortType=input  RightPortType=output  PseudoPeriodic=off  Frequencies=[]  VectorFormat=1-D array  Unit=A  AffineConversion=off
  PS-Simulink Converter5 : nesl_utility/PS-Simulink Converter  PhysicalDomain=network_engine_domain  SubClassName=ps_output  LeftPortType=input  RightPortType=output  PseudoPeriodic=off  Frequencies=[]  VectorFormat=1-D array  Unit=V  AffineConversion=off
  Simulink-PS Converter : nesl_utility/Simulink-PS Converter  PhysicalDomain=network_engine_domain  SubClassName=ps_input  LeftPortType=input  RightPortType=output  PseudoPeriodic=off  Frequencies=[]  NoiseDistribution=none  NoiseParameters=[]  Unit=V  AffineConversion=off  FilteringAndDerivatives=provide  SimscapeFilterOrder=1  InputFilterTimeConstant=0.001  UdotUserProvided=0
  Switch : fl_lib/Electrical/Electrical Elements/Switch  R_closed=1e-3 Ohm  G_open=1e-8 1/Ohm  Threshold=3  i_specify=off  i_priority=None  i=0 A  i_nominal_specify=off  i_nominal_value=1  i_nominal_unit=A  v_specify=off  v_priority=None  v=0 V  v_nominal_specify=off  v_nominal_value=1  v_nominal_unit=V
  Voltage Sensor : fl_lib/Electrical/Electrical Sensors/Voltage Sensor
  Voltage Sensor1 : fl_lib/Electrical/Electrical Sensors/Voltage Sensor
  D : PMIOPort  Side=Left
  S : PMIOPort  Port=2  Side=Right
  tag scope: device_current_41=global, device_voltage_41=global, voltage_cm_device_41=global
  wires:
  PS-Simulink Converter1/1 -> [device_voltage_41]
  PS-Simulink Converter4/1 -> [device_current_41]
  PS-Simulink Converter5/1 -> [voltage_cm_device_41]
  G/1 -> Simulink-PS Converter/1
  connections:
  Voltage Sensor/RConn2 -- Switch/RConn2 -- S/RConn1 -- Voltage Sensor1/LConn1
  Voltage Sensor/RConn1 -- PS-Simulink Converter1/LConn1
  Current Sensor/LConn1 -- Voltage Sensor/LConn1 -- D/RConn1
  Current Sensor/RConn1 -- PS-Simulink Converter4/LConn1
  PS-Simulink Converter5/LConn1 -- Voltage Sensor1/RConn1
  Voltage Sensor1/RConn2 -- Electrical Reference/LConn1
  Simulink-PS Converter/RConn1 -- Switch/RConn1
  Switch/LConn1 -- Current Sensor/RConn2

== system single_phase_multilevel_sm/flying_capacitor_leg/switch_42 ==
  G : Inport
  Current Sensor : fl_lib/Electrical/Electrical Sensors/Current Sensor
  Electrical Reference : fl_lib/Electrical/Electrical Elements/Electrical Reference
  PS-Simulink Converter1 : nesl_utility/PS-Simulink Converter  PhysicalDomain=network_engine_domain  SubClassName=ps_output  LeftPortType=input  RightPortType=output  PseudoPeriodic=off  Frequencies=[]  VectorFormat=1-D array  Unit=V  AffineConversion=off
  PS-Simulink Converter4 : nesl_utility/PS-Simulink Converter  PhysicalDomain=network_engine_domain  SubClassName=ps_output  LeftPortType=input  RightPortType=output  PseudoPeriodic=off  Frequencies=[]  VectorFormat=1-D array  Unit=A  AffineConversion=off
  PS-Simulink Converter5 : nesl_utility/PS-Simulink Converter  PhysicalDomain=network_engine_domain  SubClassName=ps_output  LeftPortType=input  RightPortType=output  PseudoPeriodic=off  Frequencies=[]  VectorFormat=1-D array  Unit=V  AffineConversion=off
  Simulink-PS Converter : nesl_utility/Simulink-PS Converter  PhysicalDomain=network_engine_domain  SubClassName=ps_input  LeftPortType=input  RightPortType=output  PseudoPeriodic=off  Frequencies=[]  NoiseDistribution=none  NoiseParameters=[]  Unit=V  AffineConversion=off  FilteringAndDerivatives=provide  SimscapeFilterOrder=1  InputFilterTimeConstant=0.001  UdotUserProvided=0
  Switch : fl_lib/Electrical/Electrical Elements/Switch  R_closed=1e-3 Ohm  G_open=1e-8 1/Ohm  Threshold=3  i_specify=off  i_priority=None  i=0 A  i_nominal_specify=off  i_nominal_value=1  i_nominal_unit=A  v_specify=off  v_priority=None  v=0 V  v_nominal_specify=off  v_nominal_value=1  v_nominal_unit=V
  Voltage Sensor : fl_lib/Electrical/Electrical Sensors/Voltage Sensor
  Voltage Sensor1 : fl_lib/Electrical/Electrical Sensors/Voltage Sensor
  D : PMIOPort  Side=Left
  S : PMIOPort  Port=2  Side=Right
  tag scope: device_current_42=global, device_voltage_42=global, voltage_cm_device_42=global
  wires:
  PS-Simulink Converter1/1 -> [device_voltage_42]
  PS-Simulink Converter4/1 -> [device_current_42]
  PS-Simulink Converter5/1 -> [voltage_cm_device_42]
  G/1 -> Simulink-PS Converter/1
  connections:
  Voltage Sensor/RConn1 -- PS-Simulink Converter1/LConn1
  S/RConn1 -- Voltage Sensor1/LConn1 -- Switch/RConn2 -- Voltage Sensor/RConn2
  Current Sensor/LConn1 -- Voltage Sensor/LConn1 -- D/RConn1
  Current Sensor/RConn1 -- PS-Simulink Converter4/LConn1
  PS-Simulink Converter5/LConn1 -- Voltage Sensor1/RConn1
  Voltage Sensor1/RConn2 -- Electrical Reference/LConn1
  Simulink-PS Converter/RConn1 -- Switch/RConn1
  Switch/LConn1 -- Current Sensor/RConn2

== system single_phase_multilevel_sm/flying_capacitor_leg/switch_51 ==
  G : Inport
  Current Sensor : fl_lib/Electrical/Electrical Sensors/Current Sensor
  Electrical Reference : fl_lib/Electrical/Electrical Elements/Electrical Reference
  PS-Simulink Converter1 : nesl_utility/PS-Simulink Converter  PhysicalDomain=network_engine_domain  SubClassName=ps_output  LeftPortType=input  RightPortType=output  PseudoPeriodic=off  Frequencies=[]  VectorFormat=1-D array  Unit=V  AffineConversion=off
  PS-Simulink Converter4 : nesl_utility/PS-Simulink Converter  PhysicalDomain=network_engine_domain  SubClassName=ps_output  LeftPortType=input  RightPortType=output  PseudoPeriodic=off  Frequencies=[]  VectorFormat=1-D array  Unit=A  AffineConversion=off
  PS-Simulink Converter5 : nesl_utility/PS-Simulink Converter  PhysicalDomain=network_engine_domain  SubClassName=ps_output  LeftPortType=input  RightPortType=output  PseudoPeriodic=off  Frequencies=[]  VectorFormat=1-D array  Unit=V  AffineConversion=off
  Simulink-PS Converter : nesl_utility/Simulink-PS Converter  PhysicalDomain=network_engine_domain  SubClassName=ps_input  LeftPortType=input  RightPortType=output  PseudoPeriodic=off  Frequencies=[]  NoiseDistribution=none  NoiseParameters=[]  Unit=V  AffineConversion=off  FilteringAndDerivatives=provide  SimscapeFilterOrder=1  InputFilterTimeConstant=0.001  UdotUserProvided=0
  Switch : fl_lib/Electrical/Electrical Elements/Switch  R_closed=1e-3 Ohm  G_open=1e-8 1/Ohm  Threshold=3  i_specify=off  i_priority=None  i=0 A  i_nominal_specify=off  i_nominal_value=1  i_nominal_unit=A  v_specify=off  v_priority=None  v=0 V  v_nominal_specify=off  v_nominal_value=1  v_nominal_unit=V
  Voltage Sensor : fl_lib/Electrical/Electrical Sensors/Voltage Sensor
  Voltage Sensor1 : fl_lib/Electrical/Electrical Sensors/Voltage Sensor
  D : PMIOPort  Side=Left
  S : PMIOPort  Port=2  Side=Right
  tag scope: device_current_51=global, device_voltage_51=global, voltage_cm_device_51=global
  wires:
  PS-Simulink Converter1/1 -> [device_voltage_51]
  PS-Simulink Converter4/1 -> [device_current_51]
  PS-Simulink Converter5/1 -> [voltage_cm_device_51]
  G/1 -> Simulink-PS Converter/1
  connections:
  Voltage Sensor/RConn1 -- PS-Simulink Converter1/LConn1
  D/RConn1 -- Voltage Sensor/LConn1 -- Current Sensor/LConn1
  Voltage Sensor/RConn2 -- Switch/RConn2 -- S/RConn1 -- Voltage Sensor1/LConn1
  Switch/LConn1 -- Current Sensor/RConn2
  Current Sensor/RConn1 -- PS-Simulink Converter4/LConn1
  Voltage Sensor1/RConn2 -- Electrical Reference/LConn1
  PS-Simulink Converter5/LConn1 -- Voltage Sensor1/RConn1
  Simulink-PS Converter/RConn1 -- Switch/RConn1

== system single_phase_multilevel_sm/flying_capacitor_leg/switch_52 ==
  G : Inport
  Current Sensor : fl_lib/Electrical/Electrical Sensors/Current Sensor
  Electrical Reference : fl_lib/Electrical/Electrical Elements/Electrical Reference
  PS-Simulink Converter1 : nesl_utility/PS-Simulink Converter  PhysicalDomain=network_engine_domain  SubClassName=ps_output  LeftPortType=input  RightPortType=output  PseudoPeriodic=off  Frequencies=[]  VectorFormat=1-D array  Unit=V  AffineConversion=off
  PS-Simulink Converter4 : nesl_utility/PS-Simulink Converter  PhysicalDomain=network_engine_domain  SubClassName=ps_output  LeftPortType=input  RightPortType=output  PseudoPeriodic=off  Frequencies=[]  VectorFormat=1-D array  Unit=A  AffineConversion=off
  PS-Simulink Converter5 : nesl_utility/PS-Simulink Converter  PhysicalDomain=network_engine_domain  SubClassName=ps_output  LeftPortType=input  RightPortType=output  PseudoPeriodic=off  Frequencies=[]  VectorFormat=1-D array  Unit=V  AffineConversion=off
  Simulink-PS Converter : nesl_utility/Simulink-PS Converter  PhysicalDomain=network_engine_domain  SubClassName=ps_input  LeftPortType=input  RightPortType=output  PseudoPeriodic=off  Frequencies=[]  NoiseDistribution=none  NoiseParameters=[]  Unit=V  AffineConversion=off  FilteringAndDerivatives=provide  SimscapeFilterOrder=1  InputFilterTimeConstant=0.001  UdotUserProvided=0
  Switch : fl_lib/Electrical/Electrical Elements/Switch  R_closed=1e-3 Ohm  G_open=1e-8 1/Ohm  Threshold=3  i_specify=off  i_priority=None  i=0 A  i_nominal_specify=off  i_nominal_value=1  i_nominal_unit=A  v_specify=off  v_priority=None  v=0 V  v_nominal_specify=off  v_nominal_value=1  v_nominal_unit=V
  Voltage Sensor : fl_lib/Electrical/Electrical Sensors/Voltage Sensor
  Voltage Sensor1 : fl_lib/Electrical/Electrical Sensors/Voltage Sensor
  D : PMIOPort  Side=Left
  S : PMIOPort  Port=2  Side=Right
  tag scope: device_current_52=global, device_voltage_52=global, voltage_cm_device_52=global
  wires:
  PS-Simulink Converter1/1 -> [device_voltage_52]
  PS-Simulink Converter4/1 -> [device_current_52]
  PS-Simulink Converter5/1 -> [voltage_cm_device_52]
  G/1 -> Simulink-PS Converter/1
  connections:
  Voltage Sensor/RConn2 -- Switch/RConn2 -- S/RConn1 -- Voltage Sensor1/LConn1
  Voltage Sensor/RConn1 -- PS-Simulink Converter1/LConn1
  Current Sensor/LConn1 -- Voltage Sensor/LConn1 -- D/RConn1
  Current Sensor/RConn1 -- PS-Simulink Converter4/LConn1
  PS-Simulink Converter5/LConn1 -- Voltage Sensor1/RConn1
  Voltage Sensor1/RConn2 -- Electrical Reference/LConn1
  Simulink-PS Converter/RConn1 -- Switch/RConn1
  Switch/LConn1 -- Current Sensor/RConn2

== system single_phase_multilevel_sm/flying_capacitor_leg/vm ==
  CFi_HF_5 : fl_lib/Electrical/Electrical Elements/Capacitor  c=CFi_HF_5 F  r=1e-6 Ohm  g=0 1/Ohm  i_specify=off  i_priority=None  i=0 A  i_nominal_specify=off  i_nominal_value=1  i_nominal_unit=A  v_specify=off  v_priority=None  v=0 V  v_nominal_specify=off  v_nominal_value=1  v_nominal_unit=V  vc_specify=on  vc_priority=High  vc=VCFc_5_init V  vc_nominal_specify=off  vc_nominal_value=1  vc_nominal_unit=V
  PS-Simulink Converter2 : nesl_utility/PS-Simulink Converter  PhysicalDomain=network_engine_domain  SubClassName=ps_output  LeftPortType=input  RightPortType=output  PseudoPeriodic=off  Frequencies=[]  VectorFormat=1-D array  Unit=V  AffineConversion=off
  Voltage Sensor1 : fl_lib/Electrical/Electrical Sensors/Voltage Sensor
  1 : PMIOPort  Side=Left
  2 : PMIOPort  Port=2  Side=Right
  tag scope: voltage_flying_capacitor_5=global
  wires:
  PS-Simulink Converter2/1 -> [voltage_flying_capacitor_5]
  connections:
  Voltage Sensor1/RConn2 -- CFi_HF_5/RConn1 -- 2/RConn1
  Voltage Sensor1/RConn1 -- PS-Simulink Converter2/LConn1
  Voltage Sensor1/LConn1 -- CFi_HF_5/LConn1 -- 1/RConn1

== system single_phase_multilevel_sm/output_filter/instantaneus_power ==
  vout : Inport
  iout : Inport  Port=2
  Product : Product
  To Workspace3 : ToWorkspace  VariableName=vout_rms_sim  SampleTime=ts
      settings: MaxDataPoints=Ns
  To Workspace4 : ToWorkspace  VariableName=iout_rms_sim  SampleTime=ts
      settings: MaxDataPoints=Ns
  To Workspace7 : ToWorkspace  VariableName=Pout_avg_sim  SampleTime=ts
      settings: MaxDataPoints=Ns
  mavg_1 : Subsystem
  rms&power : Scope  NumInputPorts=3
      settings: SampleTime=ts  ActiveDisplayYMinimum=-2.0564560895277128E-13  ActiveDisplayYMaximum=1.8508104806002774E-12
  rms2 : Subsystem
  rms3 : Subsystem
  tag scope: inverter_current_output=global, inverter_voltage_output=global
  wires:
  rms2/1(Out1) -> rms&power/1, To Workspace3/1  "vout_rms"
  rms3/1(Out1) -> rms&power/3, To Workspace4/1  "iout_rms"
  vout/1 -> [inverter_voltage_output], rms2/1(vout), Product/1
  iout/1 -> [inverter_current_output], rms3/1(iout), Product/2
  Product/1 -> mavg_1/1(in)
  mavg_1/1(out) -> rms&power/2, To Workspace7/1  "pout_mean"

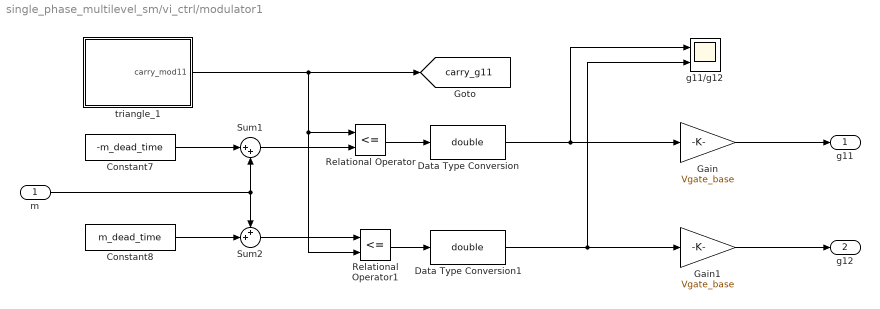
== system single_phase_multilevel_sm/vi_ctrl/modulator1 ==
  m : Inport
  Constant7 : Constant  Value=-m_dead_time
  Constant8 : Constant  Value=m_dead_time
  Data Type Conversion : DataTypeConversion  OutDataTypeStr=double  SaturateOnIntegerOverflow=off  RndMeth=Floor
  Data Type Conversion1 : DataTypeConversion  OutDataTypeStr=double  SaturateOnIntegerOverflow=off  RndMeth=Floor
  Gain : Gain  Gain=Vgate_base
  Gain1 : Gain  Gain=Vgate_base
  Relational Operator : RelationalOperator  Operator=<=
  Relational Operator1 : RelationalOperator  Operator=<=
  Sum1 : Sum  Inputs=|++
  Sum2 : Sum  Inputs=++|
  g11/g12 : Scope  NumInputPorts=2
      settings: SampleTime=tc  ActiveDisplayYMinimum=-0.12499999999999997  ActiveDisplayYMaximum=1.125
  triangle_1 : Subsystem
  g11 : Outport
  g12 : Outport  Port=2
  tag scope: carry_g11=global
  wires:
  m/1 -> Sum1/2, Sum2/1
  Relational Operator/1 -> Data Type Conversion/1
  Relational Operator1/1 -> Data Type Conversion1/1
  Data Type Conversion/1 -> g11/g12/1, Gain/1
  triangle_1/1(carry_mod11) -> Relational Operator1/2, Relational Operator/1, [carry_g11]
  Constant7/1 -> Sum1/1
  Data Type Conversion1/1 -> g11/g12/2, Gain1/1
  Sum2/1 -> Relational Operator1/1
  Constant8/1 -> Sum2/2
  Sum1/1 -> Relational Operator/2
  Gain/1 -> g11/1
  Gain1/1 -> g12/1

== system single_phase_multilevel_sm/vi_ctrl/modulator2 ==
  m : Inport
  Constant7 : Constant  Value=-m_dead_time
  Constant8 : Constant  Value=m_dead_time
  Data Type Conversion : DataTypeConversion  OutDataTypeStr=double  SaturateOnIntegerOverflow=off  RndMeth=Floor
  Data Type Conversion1 : DataTypeConversion  OutDataTypeStr=double  SaturateOnIntegerOverflow=off  RndMeth=Floor
  Gain : Gain  Gain=Vgate_base
  Gain1 : Gain  Gain=Vgate_base
  Relational Operator : RelationalOperator  Operator=<=
  Relational Operator1 : RelationalOperator  Operator=<=
  Sum1 : Sum  Inputs=|++
  Sum2 : Sum  Inputs=++|
  triangle_1 : Subsystem
  g21 : Outport
  g22 : Outport  Port=2
  tag scope: carry_g21=global
  wires:
  Sum1/1 -> Relational Operator/2
  Constant8/1 -> Sum2/2
  Sum2/1 -> Relational Operator1/1
  Data Type Conversion1/1 -> Gain1/1
  Constant7/1 -> Sum1/1
  triangle_1/1(carry_mod21) -> [carry_g21], Relational Operator1/2, Relational Operator/1
  Data Type Conversion/1 -> Gain/1
  Relational Operator1/1 -> Data Type Conversion1/1
  Relational Operator/1 -> Data Type Conversion/1
  m/1 -> Sum2/1, Sum1/2
  Gain/1 -> g21/1
  Gain1/1 -> g22/1

== system single_phase_multilevel_sm/vi_ctrl/modulator3 ==
  m : Inport
  Constant7 : Constant  Value=-m_dead_time
  Constant8 : Constant  Value=m_dead_time
  Data Type Conversion : DataTypeConversion  OutDataTypeStr=double  SaturateOnIntegerOverflow=off  RndMeth=Floor
  Data Type Conversion1 : DataTypeConversion  OutDataTypeStr=double  SaturateOnIntegerOverflow=off  RndMeth=Floor
  Gain : Gain  Gain=Vgate_base
  Gain1 : Gain  Gain=Vgate_base
  Relational Operator : RelationalOperator  Operator=<=
  Relational Operator1 : RelationalOperator  Operator=<=
  Sum1 : Sum  Inputs=|++
  Sum2 : Sum  Inputs=++|
  triangle_1 : Subsystem
  g21 : Outport
  g22 : Outport  Port=2
  tag scope: carry_g31=global
  wires:
  m/1 -> Sum1/2, Sum2/1
  Relational Operator/1 -> Data Type Conversion/1
  Relational Operator1/1 -> Data Type Conversion1/1
  Data Type Conversion/1 -> Gain/1
  triangle_1/1(carry_mod21) -> Relational Operator/1, Relational Operator1/2, [carry_g31]
  Constant7/1 -> Sum1/1
  Data Type Conversion1/1 -> Gain1/1
  Sum2/1 -> Relational Operator1/1
  Constant8/1 -> Sum2/2
  Sum1/1 -> Relational Operator/2
  Gain/1 -> g21/1
  Gain1/1 -> g22/1

== system single_phase_multilevel_sm/vi_ctrl/modulator4 ==
  m : Inport
  Constant7 : Constant  Value=-m_dead_time
  Constant8 : Constant  Value=m_dead_time
  Data Type Conversion : DataTypeConversion  OutDataTypeStr=double  SaturateOnIntegerOverflow=off  RndMeth=Floor
  Data Type Conversion1 : DataTypeConversion  OutDataTypeStr=double  SaturateOnIntegerOverflow=off  RndMeth=Floor
  Gain : Gain  Gain=Vgate_base
  Gain1 : Gain  Gain=Vgate_base
  Relational Operator : RelationalOperator  Operator=<=
  Relational Operator1 : RelationalOperator  Operator=<=
  Sum1 : Sum  Inputs=|++
  Sum2 : Sum  Inputs=++|
  triangle_1 : Subsystem
  g21 : Outport
  g22 : Outport  Port=2
  tag scope: carry_g41=global
  wires:
  m/1 -> Sum1/2, Sum2/1
  Relational Operator/1 -> Data Type Conversion/1
  Relational Operator1/1 -> Data Type Conversion1/1
  Data Type Conversion/1 -> Gain/1
  triangle_1/1(carry_mod21) -> Relational Operator/1, Relational Operator1/2, [carry_g41]
  Constant7/1 -> Sum1/1
  Data Type Conversion1/1 -> Gain1/1
  Sum2/1 -> Relational Operator1/1
  Constant8/1 -> Sum2/2
  Sum1/1 -> Relational Operator/2
  Gain/1 -> g21/1
  Gain1/1 -> g22/1

== system single_phase_multilevel_sm/vi_ctrl/modulator5 ==
  m : Inport
  Constant7 : Constant  Value=-m_dead_time
  Constant8 : Constant  Value=m_dead_time
  Data Type Conversion : DataTypeConversion  OutDataTypeStr=double  SaturateOnIntegerOverflow=off  RndMeth=Floor
  Data Type Conversion1 : DataTypeConversion  OutDataTypeStr=double  SaturateOnIntegerOverflow=off  RndMeth=Floor
  Gain : Gain  Gain=Vgate_base
  Gain1 : Gain  Gain=Vgate_base
  Relational Operator : RelationalOperator  Operator=<=
  Relational Operator1 : RelationalOperator  Operator=<=
  Sum1 : Sum  Inputs=|++
  Sum2 : Sum  Inputs=++|
  triangle_1 : Subsystem
  g21 : Outport
  g22 : Outport  Port=2
  tag scope: carry_g51=global
  wires:
  Sum1/1 -> Relational Operator/2
  Constant8/1 -> Sum2/2
  Sum2/1 -> Relational Operator1/1
  Data Type Conversion1/1 -> Gain1/1
  Constant7/1 -> Sum1/1
  triangle_1/1(carry_mod21) -> [carry_g51], Relational Operator1/2, Relational Operator/1
  Data Type Conversion/1 -> Gain/1
  Relational Operator1/1 -> Data Type Conversion1/1
  Relational Operator/1 -> Data Type Conversion/1
  m/1 -> Sum2/1, Sum1/2
  Gain/1 -> g21/1
  Gain1/1 -> g22/1

== system single_phase_multilevel_sm/vi_ctrl/pre-charge ==
  dm_in : Inport
  Ramp : simulink/Sources/Ramp  slope=-1  start=0  InitialOutput=0.5
  Saturation : Saturate  UpperLimit=0.25  LowerLimit=0
  Step1 : Step  Time=time_pwm_enable  SampleTime=0
  Switch : Switch  Criteria=u2 > Threshold  Threshold=0.5  SaturateOnIntegerOverflow=off  InputSameDT=off
  dm_out : Outport
  wires:
  Switch/1 -> dm_out/1
  ? -> Saturation/1
  Saturation/1 -> Switch/3
  dm_in/1 -> Switch/1
  Step1/1 -> Switch/2
